simulink model "drone_plant_wp1"  (R2025a)
settings: Solver=VariableStepAuto  StartTime=0.0  StopTime=100  RelTol=1e-3
settings Model: Creator=flore  LastModifiedBy=flore

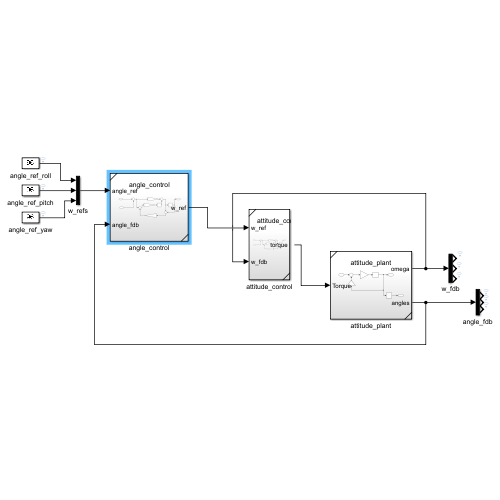
[thumbnail: Simulink's stored preview of the top-level diagram]
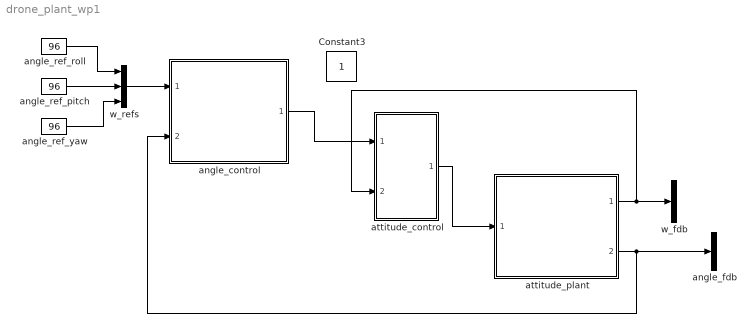
== system drone_plant_wp1 ==
  angle_control : Subsystem  ReferencedSubsystem=angle_control
  angle_fdb : Demux  Outputs=3
  angle_ref_pitch : Constant  Value=96
  angle_ref_roll : Constant  Value=96
  angle_ref_yaw : Constant  Value=96
  attitude_control : Subsystem  ReferencedSubsystem=attitude_control
  attitude_plant : Subsystem  ReferencedSubsystem=attitude_plant
  w_fdb : Demux  Outputs=3
  w_refs : Mux  Inputs=3
  Constant3 : Constant  IOType=siggen
  wires:
  attitude_plant/1 -> attitude_control/2, w_fdb/1
  attitude_plant/2 -> angle_control/2, angle_fdb/1
  angle_ref_roll/1 -> w_refs/1
  attitude_control/1 -> attitude_plant/1
  angle_ref_pitch/1 -> w_refs/2
  angle_ref_yaw/1 -> w_refs/3
  angle_control/1 -> attitude_control/1
  w_refs/1 -> angle_control/1
